simulink model "servo_hub_example"  (R2023a)
settings: Solver=FixedStepDiscrete  StartTime=0.0  StopTime=10.0  FixedStep=1e-5  RelTol=1e-3  EnableMultiTasking=on
model workspace (MATLAB code in the model file):
  | cmdLim = Simulink.Parameter;
  | cmdLim.Value = 15;
  | cmdLim.Description = 'Limit for controlling the maximum surface command angle.';
  | cmdLim.Min = 0;
  | cmdLim.Max = 90;
  | cmdLim.DocUnits = 'deg';
  | 
  | dispGain = Simulink.Parameter;
  | dispGain.Value = 0.75;
  | dispGain.Description = 'Gain applied to the displacement error.';
  | dispGain.Min = 0;
  | dispGain.Max = [];
  | dispGain.DocUnits = 'deg/sec/deg';
  | 
  | dispLim = Simulink.Parameter;
  | dispLim.Value = 30;
  | dispLim.Description = 'Limit for controlling the maximum commanded angle.';
  | dispLim.Min = 0;
  | dispLim.Max = 180;
  | dispLim.DocUnits = 'deg';
  | 
  | intGain = Simulink.Parameter;
  | intGain.Value = 0.5;
  | intGain.Description = 'Gain applied to the integral error.';
  | intGain.Min = 0;
  | intGain.Max = [];
  | intGain.DocUnits = 'deg/sec/deg/sec';
  | 
  | intLim = Simulink.Parameter;
  | intLim.Value = 5;
  | intLim.Description = 'Limit for controlling the maximum commanded angle.';
  | intLim.Min = 0;
  | intLim.Max = 90;
  | intLim.DocUnits = 'deg';
  | 
  | rateGain = Simulink.Parameter;
  | rateGain.Value = 2;
  | rateGain.Description = 'Gain applied to the rate error.';
  | rateGain.Min = 0;
  | rateGain.Max = [];
  | rateGain.DocUnits = 'deg/deg/sec';
  | 
  | rateLim = Simulink.Parameter;
  | rateLim.Value = 6;
  | rateLim.Description = 'Limit for controlling the maximum commanded angle.';
  | rateLim.Min = 0;
  | rateLim.Max = 180;
  | rateLim.DocUnits = 'deg/sec';
  | 
  | hdgGain = Simulink.Parameter;
  | hdgGain.Value = 0.015;
settings Model: RequirementInfo={} %GIDa_fe9045fd_0412_4b6e_8206_617cc20e6fde  DataDictionary=model_config.sldd  Creator=Administrator  LastModifiedBy=Administrator
settings ConfigSet: Description=导出函数模型默认使用并行编译代码生成，速度更快
settings SolverCC: AlgebraicLoopSolver=TrustRegion  AutoInsertRateTranBlk=on
settings DataIOCC: SaveOutput=off  SignalLogging=off  DSMLogging=off  SaveTime=off
settings OptimizationCC: DefaultParameterBehavior=Inlined  UseDivisionForNetSlopeComputation=on  GainParamInheritBuiltInType=on  UseFloatMulNetSlope=on  DefaultUnderspecifiedDataType=single  UseSpecifiedMinMax=on  InlineInvariantSignals=on  PassReuseOutputArgsAs=Individual arguments  ZeroExternalMemoryAtStartup=off  ZeroInternalMemoryAtStartup=off  NoFixptDivByZeroProtection=on  EfficientFloat2IntCast=on  MaxStackSize=64  OptimizeBlockOrder=speed  OptimizationLevel=level1  EfficientTunableParamExpr=on
settings DebuggingCC: SignalInfNanChecking=error  CheckMatrixSingularityMsg=error  IntegerOverflowMsg=error  ParameterPrecisionLossMsg=none  UnconnectedInputMsg=error  UnconnectedOutputMsg=error  UnconnectedLineMsg=error  UniqueDataStoreMsg=error  AllowSymbolicDim=off  StrictBusMsg=ErrorOnBusTreatedAsVector  SFExecutionAtInitializationDiag=none  IntegerSaturationMsg=error  ArithmeticOperatorsInVariantConditions=warning
settings HardwareCC: ProdBitPerPointer=32  ProdBitPerSizeT=32  ProdBitPerPtrDiffT=32  ProdLargestAtomicInteger=Long  ProdLargestAtomicFloat=Double  ProdWordSize=32  ProdLongLongMode=on  ProdHWDeviceType=ARM Compatible->ARM Cortex
settings ModelReferenceCC: EnableParallelModelReferenceBuilds=on
settings SFSimCC: MATLABDynamicMemAlloc=off
settings RTWCC: Description=Embedded Coder  SystemTargetFile=ert.tlc  GenCodeOnly=on  TemplateMakefile=ert_default_tmf  GenerateReport=on  Toolchain=GNU Tools for ARM Embedded Processors  BuildConfiguration=Faster Runs  IncludeHyperlinkInReport=on  PortableWordSizes=on  GenerateTraceInfo=on  GenerateTraceReport=on  GenerateTraceReportSl=on  GenerateTraceReportSf=on  GenerateTraceReportEml=on  GenerateCodeMetricsReport=on  GenerateCodeReplacementReport=on
settings CodeAppCC: ForceParamTrailComments=on  IgnoreCustomStorageClasses=off  MaxIdLength=63  OperatorAnnotations=on  SimulinkDataObjDesc=on  SFDataObjDesc=on  MATLABFcnDesc=on  CustomSymbolStrGlobalVar=_rt_$N$M  CustomSymbolStrType=$N$M  CustomSymbolStrFcn=$N$M$F  CustomSymbolStrMacro=$N$M  InsertBlockDesc=on  StateflowObjectComments=on  MATLABSourceComments=on  EnableCustomComments=on  ReqsInCode=on
settings ERTTargetCC: TargetLangStandard=C99 (ISO)  CodeReplacementLibrary=YuanHub Math  UtilityFuncGeneration=Shared location  MultiwordLength=2048  IncludeMdlTerminateFcn=off  CombineSignalStateStructs=on  SuppressErrorStatus=on  SupportNonFinite=off  SupportComplex=off  ExtModeTransport=3  ExtModeStaticAlloc=on  ExtModeStaticAllocSize=2048  ExtModeMexFile=ext_xcp  ExtModeIntrfLevel=Level2 - Open  ERTCustomFileTemplate=example_file_process.tlc  ERTFilePackagingFormat=Compact  IndentStyle=Allman  IndentSize=4
settings ConfigComp: CovScope=ReferencedModels  CovSaveName=covdata_rollAP  CovMetricSettings=dcmtrwe  CovHTMLOptions=-sRT=1 -aTS=1 -bRG=1 -bTC=1 -hTR=1 -nFC=0 -scm=1 -bcm=1 -xEv=0  CovSaveCumulativeToWorkspaceVar=on  CovSaveSingleToWorkspaceVar=on  CovCumulativeVarName=covCumulativeData_rollAP  CovReportOnPause=off  CovExternalEMLEnable=off  CovSFcnEnable=off

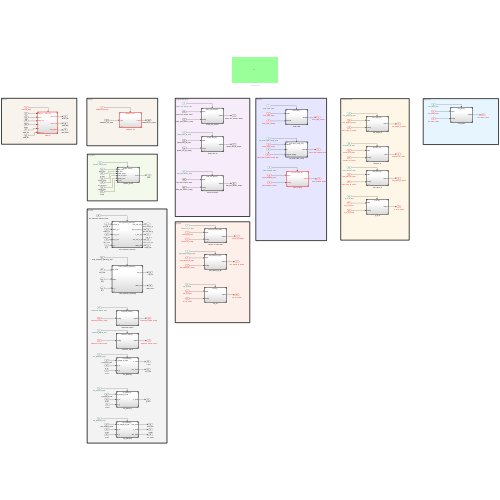
[thumbnail: Simulink's stored preview of the top-level diagram]
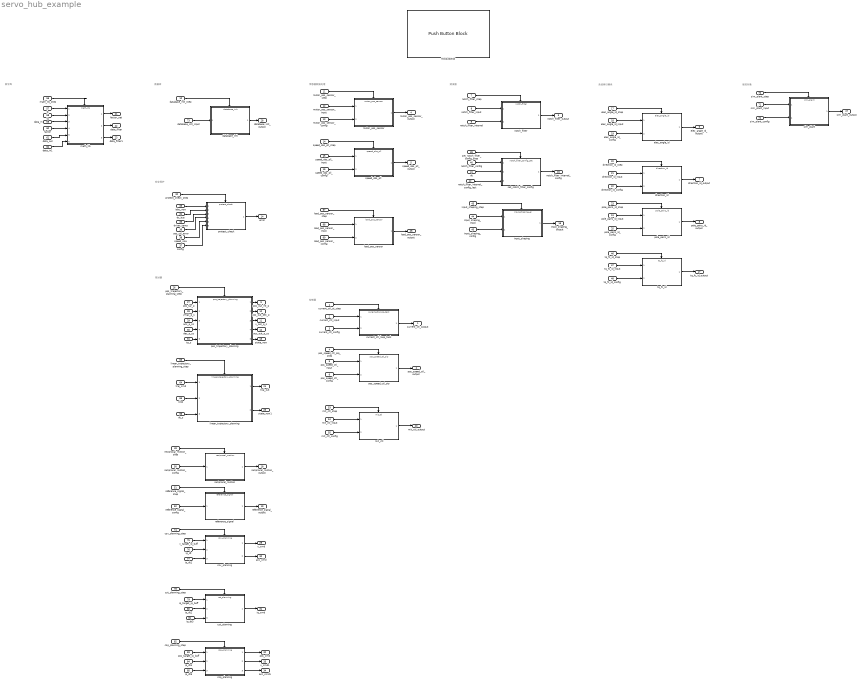
== system servo_hub_example ==
  note: 控制器
  note: 滤波器
  note: 系统辨识模块
  note: 规划器
  note: 数据库
  note: 安全保护
  note: 传感器数据处理
  note: 数学库
  note: 被控对象
  current_ctl_pi_step : Inport  SampleTime=1e-5  OutputFunctionCall=on
  current_ctl_input : Inport  Port=2  OutDataTypeStr=Bus: CurrentCtlInput  BusOutputAsStruct=on
  current_ctl_config : Inport  Port=3  OutDataTypeStr=Bus: CurrentCtlConfig  BusOutputAsStruct=on
  pos_speed_ctl_pip_step : Inport  Port=4  SampleTime=1e-5  OutputFunctionCall=on
  pos_speed_ctl_input : Inport  Port=5  OutDataTypeStr=Bus: PosSpeedCtlInput  BusOutputAsStruct=on
  pos_speed_ctl_config : Inport  Port=6  OutDataTypeStr=Bus: PosSpeedCtlConfig  BusOutputAsStruct=on
  notch_filter_step : Inport  Port=7  SampleTime=1e-5  OutputFunctionCall=on
  notch_filter_input : Inport  Port=8  OutDataTypeStr=Bus: NotchFilterInput  BusOutputAsStruct=on
  notch_filter_internal : Inport  Port=9  OutDataTypeStr=Bus: NotchFilterInternal  BusOutputAsStruct=on
  database_init_step : Inport  Port=10  SampleTime=1e-5  OutputFunctionCall=on
  motor_pos_sensor_step : Inport  Port=11  SampleTime=1e-5  OutputFunctionCall=on
  motor_pos_sensor_input : Inport  Port=12  OutDataTypeStr=Bus: MotorPosSensorInput  BusOutputAsStruct=on
  motor_pos_sensor_config : Inport  Port=13  OutDataTypeStr=Bus: MotorPosSensorConfig  BusOutputAsStruct=on
  speed_obs_pll_step : Inport  Port=14  SampleTime=1e-5  OutputFunctionCall=on
  speed_obs_pll_input : Inport  Port=15  OutDataTypeStr=Bus: SpeedObsPllInput  BusOutputAsStruct=on
  speed_obs_pll_config : Inport  Port=16  OutDataTypeStr=Bus: SpeedObsPllConfig  BusOutputAsStruct=on
  elec_angle_id_step : Inport  Port=17  SampleTime=1e-5  OutputFunctionCall=on
  elec_angle_id_input : Inport  Port=18  OutDataTypeStr=Bus: ElecAngleIdInput  BusOutputAsStruct=on
  elec_angle_id_config : Inport  Port=19  OutDataTypeStr=Bus: ElecAngleIdConfig  BusOutputAsStruct=on
  direction_id_step : Inport  Port=20  SampleTime=1e-5  OutputFunctionCall=on
  direction_id_input : Inport  Port=21  OutDataTypeStr=Bus: DirectionIdInput  BusOutputAsStruct=on
  direction_id_config : Inport  Port=22  OutDataTypeStr=Bus: DirectionIdConfig  BusOutputAsStruct=on
  pole_pairs_id_step : Inport  Port=23  SampleTime=1e-5  OutputFunctionCall=on
  pole_pairs_id_input : Inport  Port=24  OutDataTypeStr=Bus: PolePairsIdInput  BusOutputAsStruct=on
  pole_pairs_id_config : Inport  Port=25  OutDataTypeStr=Bus: PolePairsIdConfig  BusOutputAsStruct=on
  pos_trajectory_planning_step : Inport  Port=26  SampleTime=1e-5  OutputFunctionCall=on
  pos_tar_p : Inport  Port=27
  vmax_p_s : Inport  Port=28
  acc_p_ss : Inport  Port=29
  dec_p_ss : Inport  Port=30
  tp_s : Inport  Port=31
  protect_check_step : Inport  Port=32  SampleTime=1e-5  OutputFunctionCall=on
  iabc_now : Inport  Port=33
  dc_bus : Inport  Port=34
  driver_temp : Inport  Port=35
  pos_ctl_error : Inport  Port=36
  config : Inport  Port=37  OutDataTypeStr=Bus: MotorCtlSmConfig  BusOutputAsStruct=on
  speed_now : Inport  Port=38
  set_notch_filter_config_step : Inport  Port=39  SampleTime=1e-5  OutputFunctionCall=on
  notch_filter_config : Inport  Port=40  OutDataTypeStr=Bus: NotchFilterConfig  BusOutputAsStruct=on
  dt : Inport  Port=41
  notch_filter_internal_config_last : Inport  Port=42  OutDataTypeStr=Bus: NotchFilterInternal  BusOutputAsStruct=on
  input_shaping_step : Inport  Port=43  SampleTime=1e-5  OutputFunctionCall=on
  input_shaping_input : Inport  Port=44  OutDataTypeStr=Bus: InputShapingInput  BusOutputAsStruct=on
  input_shaping_config : Inport  Port=45  OutDataTypeStr=Bus: InputShapingConfig  BusOutputAsStruct=on
  tq_fc_id_step : Inport  Port=46  SampleTime=1e-5  OutputFunctionCall=on
  tq_fc_id_input : Inport  Port=47  OutDataTypeStr=Bus: TqFcIdInput  BusOutputAsStruct=on
  tq_fc_id_config : Inport  Port=48  OutDataTypeStr=Bus: TqFcIdConfig  BusOutputAsStruct=on
  reciprocal_motion_step : Inport  Port=49  SampleTime=1e-5  OutputFunctionCall=on
  reciprocal_motion_config : Inport  Port=50  OutDataTypeStr=Bus: ReciprocalMotionConfig  BusOutputAsStruct=on
  reference_signal_step : Inport  Port=51  SampleTime=1e-5  OutputFunctionCall=on
  reference_signal_config : Inport  Port=52  OutDataTypeStr=Bus: ReferenceSignalConfig  BusOutputAsStruct=on
  mit_ctl_step : Inport  Port=53  SampleTime=1e-5  OutputFunctionCall=on
  mit_ctl_input : Inport  Port=54  OutDataTypeStr=Bus: MitCtlInput  BusOutputAsStruct=on
  mit_ctl_config : Inport  Port=55  OutDataTypeStr=Bus: MitCtlConfig  BusOutputAsStruct=on
  math_lib_step : Inport  Port=56  SampleTime=1e-5  OutputFunctionCall=on
  fc : Inport  Port=57
  ts : Inport  Port=58
  data_in : Inport  Port=59
  factor : Inport  Port=60
  data_out : Inport  Port=61
  data_in1 : Inport  Port=62  OutDataTypeStr=single  PortDimensions=3
  linear_trajectory_planning_step : Inport  Port=63  SampleTime=1e-5  OutputFunctionCall=on
  traj_cmd : Inport  Port=64
  slop : Inport  Port=65
  dt_s : Inport  Port=66
  load_pos_sensor_step : Inport  Port=67  SampleTime=1e-5  OutputFunctionCall=on
  load_pos_sensor_input : Inport  Port=68  OutDataTypeStr=Bus: LoadPosSensorInput  BusOutputAsStruct=on
  load_pos_sensor_config : Inport  Port=69  OutDataTypeStr=Bus: LoadPosSensorConfig  BusOutputAsStruct=on
  sim_plant_step : Inport  Port=70  SampleTime=1e-5  OutputFunctionCall=on
  sim_plant_input : Inport  Port=71  OutDataTypeStr=Bus: SimPlantInput  BusOutputAsStruct=on
  sim_plant_config : Inport  Port=72  OutDataTypeStr=Bus: SimPlantConfig  BusOutputAsStruct=on
  database_init_input : Inport  Port=73  OutDataTypeStr=Bus: Axis  BusOutputAsStruct=on
  csv_planning_step : Inport  Port=74  SampleTime=1e-5  OutputFunctionCall=on
  v_target_ip_buff : Inport  Port=75
  ip_dt : Inport  Port=76
  ip_dt1 : Inport  Port=77
  cst_planning_step : Inport  Port=78  SampleTime=1e-5  OutputFunctionCall=on
  iq_target_ip_buff : Inport  Port=79
  ip_dt2 : Inport  Port=80
  ip_dt3 : Inport  Port=81
  csp_planning_step : Inport  Port=82  SampleTime=1e-5  OutputFunctionCall=on
  pos_target_ip_buff : Inport  Port=83
  ip_dt4 : Inport  Port=84
  ip_dt5 : Inport  Port=85
  csp_planning : ModelReference  ModelNameDialog=csp_planning.slx  SimulationMode=Normal  ModelReferenceVersion=2.504  TriggerPortName=Trigger  TriggerPortTriggerType=function-call  TriggerPortStatesWhenEnabling=held
  cst_planning : ModelReference  ModelNameDialog=cst_planning.slx  SimulationMode=Normal  ModelReferenceVersion=2.483  TriggerPortName=Trigger  TriggerPortTriggerType=function-call  TriggerPortStatesWhenEnabling=held
  csv_planning : ModelReference  ModelNameDialog=csv_planning.slx  SimulationMode=Normal  ModelReferenceVersion=2.505  TriggerPortName=Trigger  TriggerPortTriggerType=function-call  TriggerPortStatesWhenEnabling=held
  current_ctl_loop_task : ModelReference  ModelNameDialog=current_ctl_loop_task.slx  SimulationMode=Normal  ModelReferenceVersion=2.1056  TriggerPortName=Trigger  TriggerPortTriggerType=function-call  TriggerPortStatesWhenEnabling=held
  database_init : ModelReference  ModelNameDialog=database_init.slx  SimulationMode=Normal  ModelReferenceVersion=2.842  TriggerPortName=Trigger  TriggerPortTriggerType=function-call  TriggerPortStatesWhenEnabling=held
  direction_id : ModelReference  ModelNameDialog=direction_id.slx  SimulationMode=Normal  ModelReferenceVersion=2.837  TriggerPortName=Trigger  TriggerPortTriggerType=function-call  TriggerPortStatesWhenEnabling=held
  elec_angle_id : ModelReference  ModelNameDialog=elec_angle_id.slx  SimulationMode=Normal  ModelReferenceVersion=2.991  TriggerPortName=Trigger  TriggerPortTriggerType=function-call  TriggerPortStatesWhenEnabling=held
  input_shaping : ModelReference  ModelNameDialog=input_shaping_ei.slx  SimulationMode=Normal  ModelReferenceVersion=1.221  TriggerPortName=Trigger  TriggerPortTriggerType=function-call  TriggerPortStatesWhenEnabling=held
  linear_trajectory_planning : ModelReference  ModelNameDialog=linear_trajectory_planning.slx  UsingDefaultArgumentValue=0,0,0  SimulationMode=Normal  ModelReferenceVersion=2.317  TriggerPortName=Trigger  TriggerPortTriggerType=function-call  TriggerPortStatesWhenEnabling=held
  load_pos_sensor : ModelReference  ModelNameDialog=load_pos_sensor.slx  SimulationMode=Normal  ModelReferenceVersion=2.969  TriggerPortName=Trigger  TriggerPortTriggerType=function-call  TriggerPortStatesWhenEnabling=held
  math_lib : ModelReference  ModelNameDialog=math_lib.slx  SimulationMode=Normal  ModelReferenceVersion=2.867  TriggerPortName=Trigger  TriggerPortTriggerType=function-call  TriggerPortStatesWhenEnabling=held
  mit_ctl : ModelReference  ModelNameDialog=mit_ctl.slx  SimulationMode=Normal  ModelReferenceVersion=2.994  TriggerPortName=Trigger  TriggerPortTriggerType=function-call  TriggerPortStatesWhenEnabling=held
  motor_pos_sensor : ModelReference  ModelNameDialog=motor_pos_sensor.slx  SimulationMode=Normal  ModelReferenceVersion=2.961  TriggerPortName=Trigger  TriggerPortTriggerType=function-call  TriggerPortStatesWhenEnabling=held
  notch_filter : ModelReference  ModelNameDialog=notch_filter.slx  UsingDefaultArgumentValue=0,0,0,0  SimulationMode=Normal  ModelReferenceVersion=1.227  TriggerPortName=Trigger  TriggerPortTriggerType=function-call  TriggerPortStatesWhenEnabling=held
  pole_pairs_id : ModelReference  ModelNameDialog=pole_pairs_id.slx  SimulationMode=Normal  ModelReferenceVersion=2.874  TriggerPortName=Trigger  TriggerPortTriggerType=function-call  TriggerPortStatesWhenEnabling=held
  pos_speed_ctl_pip : ModelReference  ModelNameDialog=pos_speed_ctl_pip.slx  SimulationMode=Normal  ModelReferenceVersion=2.979  TriggerPortName=Trigger  TriggerPortTriggerType=function-call  TriggerPortStatesWhenEnabling=held
  pos_trajectory_planning : ModelReference  ModelNameDialog=pos_trajectory_planning.slx  SimulationMode=Normal  ModelReferenceVersion=2.53  TriggerPortName=Trigger  TriggerPortTriggerType=function-call  TriggerPortStatesWhenEnabling=held
  protect_check : ModelReference  ModelNameDialog=protect_check.slx  SimulationMode=Normal  ModelReferenceVersion=2.838  TriggerPortName=Trigger  TriggerPortTriggerType=function-call  TriggerPortStatesWhenEnabling=held
  reciprocal_motion : ModelReference  ModelNameDialog=reciprocal_motion.slx  SimulationMode=Normal  ModelReferenceVersion=2.113  TriggerPortName=Trigger  TriggerPortTriggerType=function-call  TriggerPortStatesWhenEnabling=held
  reference_signal : ModelReference  ModelNameDialog=reference_signal.slx  SimulationMode=Normal  ModelReferenceVersion=2.134  TriggerPortName=Trigger  TriggerPortTriggerType=function-call  TriggerPortStatesWhenEnabling=held
  set_notch_filter_config : ModelReference  ModelNameDialog=notch_filter_config_set.slx  UsingDefaultArgumentValue=0,0,0,0  SimulationMode=Normal  ModelReferenceVersion=1.304  TriggerPortName=Trigger  TriggerPortTriggerType=function-call  TriggerPortStatesWhenEnabling=held
  sim_plant : ModelReference  ModelNameDialog=sim_plant.slx  SimulationMode=Normal  ModelReferenceVersion=1.108  TriggerPortName=Trigger  TriggerPortTriggerType=function-call  TriggerPortStatesWhenEnabling=held
  speed_obs_pll : ModelReference  ModelNameDialog=speed_obs_pll.slx  UsingDefaultArgumentValue=0,0,0  SimulationMode=Normal  ModelReferenceVersion=2.279  TriggerPortName=Trigger  TriggerPortTriggerType=function-call  TriggerPortStatesWhenEnabling=held
  tq_fc_id : ModelReference  ModelNameDialog=tq_fc_id.slx  SimulationMode=Normal  ModelReferenceVersion=2.1145  TriggerPortName=Trigger  TriggerPortTriggerType=function-call  TriggerPortStatesWhenEnabling=held
  代码生成按钮 : PushButtonBlock  ButtonText=生成代码
      settings: OpenFcn=auto_code_gen_servo_hub_example
  current_ctl_output : Outport  OutDataTypeStr=Bus: CurrentCtlOutput
  pos_speed_ctl_output : Outport  Port=2  OutDataTypeStr=Bus: PosSpeedCtlOutput
  notch_filter_output : Outport  Port=3  OutDataTypeStr=Bus: NotchFilterOutput
  motor_pos_sensor_output : Outport  Port=4  OutDataTypeStr=Bus: MotorPosSensorOutput
  speed_obs_pll_output : Outport  Port=5  OutDataTypeStr=Bus: SpeedObsPllOutput
  elec_angle_id_output : Outport  Port=6  OutDataTypeStr=Bus: ElecAngleIdOutput
  direction_id_output : Outport  Port=7  OutDataTypeStr=Bus: DirectionIdOutput
  pole_pairs_id_output : Outport  Port=8  OutDataTypeStr=Bus: PolePairsIdOutput
  pos_out_int_p : Outport  Port=9
  pos_out_dec_p : Outport  Port=10
  v_out_p_s : Outport  Port=11
  acc_out_p_ss : Outport  Port=12
  state_now : Outport  Port=13
  error : Outport  Port=14
  notch_filter_internal_config : Outport  Port=15  OutDataTypeStr=Bus: NotchFilterInternal
  input_shaping_output : Outport  Port=16  OutDataTypeStr=Bus: InputShapingOutput
  tq_fc_id_output : Outport  Port=17  OutDataTypeStr=Bus: TqFcIdOutput
  reciprocal_motion_output : Outport  Port=18  OutDataTypeStr=Bus: ReciprocalMotionOutput
  reference_signal_output : Outport  Port=19  OutDataTypeStr=Bus: ReferenceSignalOutput
  mit_ctl_output : Outport  Port=20  OutDataTypeStr=Bus: MitCtlOutput
  factor_set : Outport  Port=21
  data_filter : Outport  Port=22
  data_filter1 : Outport  Port=23
  traj_out : Outport  Port=24
  state_now1 : Outport  Port=25
  load_pos_sensor_output : Outport  Port=26  OutDataTypeStr=Bus: LoadPosSensorOutput
  sim_plant_output : Outport  Port=27  OutDataTypeStr=Bus: SimPlantOutput
  database_init_output : Outport  Port=28  OutDataTypeStr=Bus: Axis
  v_cmd : Outport  Port=29
  acc_cmd : Outport  Port=30
  iq_cmd : Outport  Port=31
  pos_cmd : Outport  Port=32
  v_cmd1 : Outport  Port=33
  acc_cmd1 : Outport  Port=34
  wires:
  current_ctl_pi_step/1 -> current_ctl_loop_task/Trigger
  current_ctl_input/1 -> current_ctl_loop_task/1
  current_ctl_config/1 -> current_ctl_loop_task/2
  current_ctl_loop_task/1 -> current_ctl_output/1
  pos_speed_ctl_pip_step/1 -> pos_speed_ctl_pip/Trigger
  pos_speed_ctl_input/1 -> pos_speed_ctl_pip/1
  pos_speed_ctl_config/1 -> pos_speed_ctl_pip/2
  pos_speed_ctl_pip/1 -> pos_speed_ctl_output/1
  notch_filter_step/1 -> notch_filter/Trigger
  notch_filter/1 -> notch_filter_output/1
  notch_filter_internal/1 -> notch_filter/2
  notch_filter_input/1 -> notch_filter/1
  database_init_step/1 -> database_init/Trigger
  motor_pos_sensor_input/1 -> motor_pos_sensor/1
  motor_pos_sensor_config/1 -> motor_pos_sensor/2
  motor_pos_sensor/1 -> motor_pos_sensor_output/1
  speed_obs_pll/1 -> speed_obs_pll_output/1
  speed_obs_pll_input/1 -> speed_obs_pll/1
  speed_obs_pll_step/1 -> speed_obs_pll/Trigger
  speed_obs_pll_config/1 -> speed_obs_pll/2
  elec_angle_id_config/1 -> elec_angle_id/2
  elec_angle_id/1 -> elec_angle_id_output/1
  elec_angle_id_input/1 -> elec_angle_id/1
  elec_angle_id_step/1 -> elec_angle_id/Trigger
  direction_id_step/1 -> direction_id/Trigger
  direction_id_input/1 -> direction_id/1
  direction_id/1 -> direction_id_output/1
  direction_id_config/1 -> direction_id/2
  pole_pairs_id/1 -> pole_pairs_id_output/1
  pole_pairs_id_input/1 -> pole_pairs_id/1
  pole_pairs_id_step/1 -> pole_pairs_id/Trigger
  pole_pairs_id_config/1 -> pole_pairs_id/2
  tp_s/1 -> pos_trajectory_planning/5
  pos_trajectory_planning/2 -> pos_out_dec_p/1
  dec_p_ss/1 -> pos_trajectory_planning/4
  acc_p_ss/1 -> pos_trajectory_planning/3
  pos_trajectory_planning/5 -> state_now/1
  pos_trajectory_planning/1 -> pos_out_int_p/1
  pos_trajectory_planning/3 -> v_out_p_s/1
  pos_tar_p/1 -> pos_trajectory_planning/1
  vmax_p_s/1 -> pos_trajectory_planning/2
  pos_trajectory_planning/4 -> acc_out_p_ss/1
  pos_trajectory_planning_step/1 -> pos_trajectory_planning/Trigger
  protect_check_step/1 -> protect_check/Trigger
  iabc_now/1 -> protect_check/1
  dc_bus/1 -> protect_check/2
  driver_temp/1 -> protect_check/3
  pos_ctl_error/1 -> protect_check/4
  protect_check/1 -> error/1
  set_notch_filter_config/1 -> notch_filter_internal_config/1
  notch_filter_config/1 -> set_notch_filter_config/1
  set_notch_filter_config_step/1 -> set_notch_filter_config/Trigger
  dt/1 -> set_notch_filter_config/2
  notch_filter_internal_config_last/1 -> set_notch_filter_config/3
  input_shaping_config/1 -> input_shaping/2
  input_shaping/1 -> input_shaping_output/1
  input_shaping_step/1 -> input_shaping/Trigger
  input_shaping_input/1 -> input_shaping/1
  tq_fc_id_input/1 -> tq_fc_id/1
  tq_fc_id/1 -> tq_fc_id_output/1
  tq_fc_id_step/1 -> tq_fc_id/Trigger
  tq_fc_id_config/1 -> tq_fc_id/2
  motor_pos_sensor_step/1 -> motor_pos_sensor/Trigger
  reciprocal_motion/1 -> reciprocal_motion_output/1
  reciprocal_motion_config/1 -> reciprocal_motion/1
  reciprocal_motion_step/1 -> reciprocal_motion/Trigger
  reference_signal_config/1 -> reference_signal/1
  reference_signal/1 -> reference_signal_output/1
  reference_signal_step/1 -> reference_signal/Trigger
  mit_ctl/1 -> mit_ctl_output/1
  mit_ctl_config/1 -> mit_ctl/2
  mit_ctl_input/1 -> mit_ctl/1
  mit_ctl_step/1 -> mit_ctl/Trigger
  math_lib/1 -> factor_set/1
  ts/1 -> math_lib/2
  fc/1 -> math_lib/1
  factor/1 -> math_lib/4
  data_in/1 -> math_lib/3
  data_out/1 -> math_lib/5
  math_lib/2 -> data_filter/1
  math_lib_step/1 -> math_lib/Trigger
  data_in1/1 -> math_lib/6
  math_lib/3 -> data_filter1/1
  linear_trajectory_planning_step/1 -> linear_trajectory_planning/Trigger
  traj_cmd/1 -> linear_trajectory_planning/1
  slop/1 -> linear_trajectory_planning/2
  dt_s/1 -> linear_trajectory_planning/3
  linear_trajectory_planning/1 -> traj_out/1
  linear_trajectory_planning/2 -> state_now1/1
  load_pos_sensor_input/1 -> load_pos_sensor/1
  load_pos_sensor/1 -> load_pos_sensor_output/1
  load_pos_sensor_step/1 -> load_pos_sensor/Trigger
  load_pos_sensor_config/1 -> load_pos_sensor/2
  sim_plant_input/1 -> sim_plant/1
  sim_plant_config/1 -> sim_plant/2
  sim_plant/1 -> sim_plant_output/1
  sim_plant_step/1 -> sim_plant/Trigger
  database_init/1 -> database_init_output/1
  database_init_input/1 -> database_init/1
  config/1 -> protect_check/6
  speed_now/1 -> protect_check/5
  csv_planning_step/1 -> csv_planning/Trigger
  v_target_ip_buff/1 -> csv_planning/1
  ip_dt/1 -> csv_planning/2
  ip_dt1/1 -> csv_planning/3
  csv_planning/1 -> v_cmd/1
  csv_planning/2 -> acc_cmd/1
  ip_dt3/1 -> cst_planning/3
  iq_target_ip_buff/1 -> cst_planning/1
  cst_planning/1 -> iq_cmd/1
  cst_planning_step/1 -> cst_planning/Trigger
  ip_dt2/1 -> cst_planning/2
  ip_dt5/1 -> csp_planning/3
  csp_planning/2 -> v_cmd1/1
  pos_target_ip_buff/1 -> csp_planning/1
  csp_planning/1 -> pos_cmd/1
  csp_planning_step/1 -> csp_planning/Trigger
  ip_dt4/1 -> csp_planning/2
  csp_planning/3 -> acc_cmd1/1
